simulink model "Proyecto"  (R2023a)
settings: Solver=ode15s  StartTime=0.0  StopTime=10  MaxStep=1E-3  RelTol=1e-3
libraries: fl_lib x16, nesl_utility x6, slpidlib x1
settings Model: LastModifiedBy=DELL
settings DataIOCC: SaveFormat=Array  ReturnWorkspaceOutputs=off  TimeSaveName=t
settings DebuggingCC: AlgebraicLoopMsg=none  ArtificialAlgebraicLoopMsg=none  MaxConsecutiveZCsMsg=none  ModelReferenceExtraNoncontSigs=none  OperatingPointInterfaceChecksumMismatchMsg=none
settings RTWCC: GPUComputeCapability=5.0

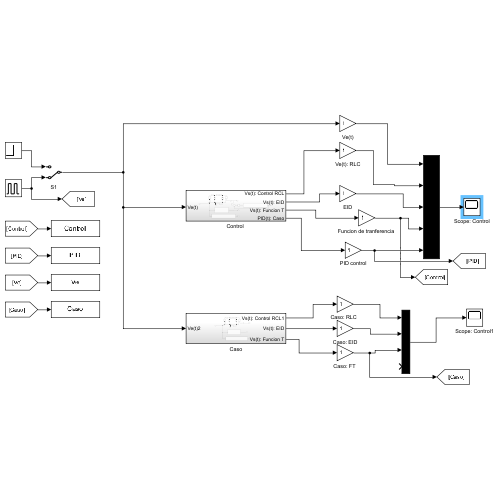
[thumbnail: Simulink's stored preview of the top-level diagram]
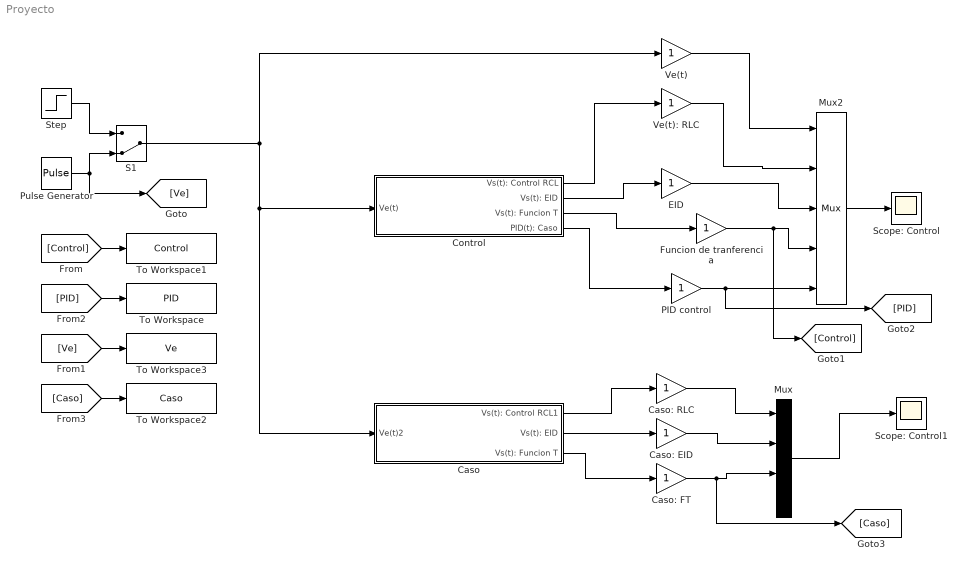
== system Proyecto ==
  Caso : Subsystem
  Caso: EID : Gain
  "Caso: FT " : Gain
  "Caso: RLC  " : Gain
  "Control " : Subsystem
  EID : Gain
  "Funcion de tranferencia " : Gain
  Mux : Mux
  Mux2 : Mux  Inputs=5
  PID control : Gain
  Pulse Generator : DiscretePulseGenerator  PulseType=Time based  Period=10  PulseWidth=10  PhaseDelay=1
  S1 : ManualSwitch  CurrentSetting=0
  Scope: Control : Scope
  Scope: Control1 : Scope
  Step : Step  SampleTime=0
  To Workspace : ToWorkspace  VariableName=PID  SampleTime=-1
  To Workspace1 : ToWorkspace  VariableName=Control  SampleTime=-1
  To Workspace2 : ToWorkspace  VariableName=Caso  SampleTime=-1
  To Workspace3 : ToWorkspace  VariableName=Ve  SampleTime=-1
  Ve(t) : Gain
  Ve(t): RLC : Gain
  wires:
  Mux2/1 -> Scope: Control/1
  Step/1 -> S1/1
  "Control "/1(Vs(t): Control RCL) -> Ve(t): RLC/1
  Pulse Generator/1 -> S1/2, [Ve]
  S1/1 -> Caso/1(Ve(t)2), "Control "/1(Ve(t)), Ve(t)/1
  "Control "/2(Vs(t): EID) -> EID/1
  EID/1 -> Mux2/3
  "Control "/3(Vs(t): Funcion T) -> "Funcion de tranferencia "/1
  "Funcion de tranferencia "/1 -> [Control], Mux2/4
  Ve(t)/1 -> Mux2/1
  Ve(t): RLC/1 -> Mux2/2
  Caso/1(Vs(t): Control RCL1) -> "Caso: RLC  "/1
  Mux/1 -> Scope: Control1/1
  Caso/2(Vs(t): EID) -> Caso: EID/1
  Caso/3(Vs(t): Funcion T) -> "Caso: FT "/1
  "Caso: RLC  "/1 -> Mux/1
  Caso: EID/1 -> Mux/2
  "Caso: FT "/1 -> [Caso], Mux/3
  [Control] -> To Workspace1/1
  [Ve] -> To Workspace3/1
  [PID] -> To Workspace/1
  [Caso] -> To Workspace2/1
  "Control "/4(PID(t): Caso) -> PID control/1
  PID control/1 -> [PID], Mux2/5

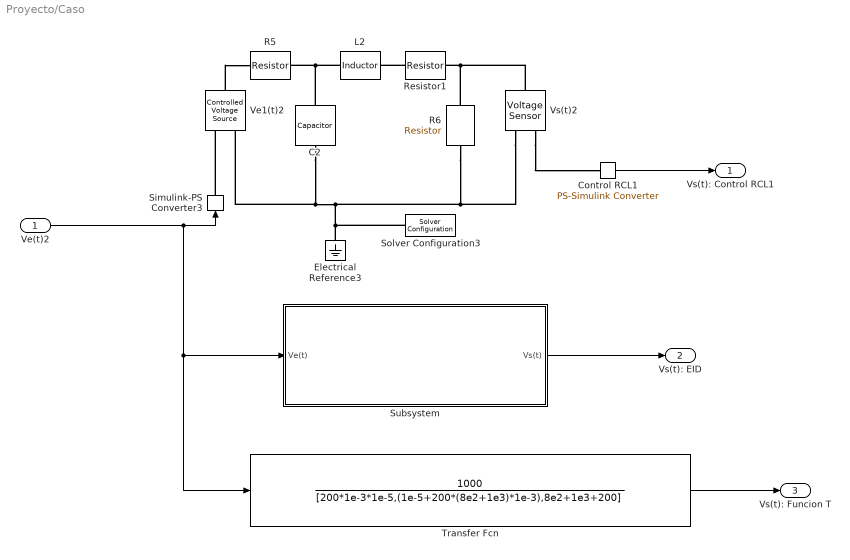
== system Proyecto/Caso ==
  Ve(t)2 : Inport
  C2 : fl_lib/Electrical/Electrical Elements/Capacitor  c=1e-3 F  r=1e-6 Ohm  g=0 1/Ohm  i_specify=off  i_priority=None  i=0 A  i_nominal_specify=off  i_nominal_unit=A  i_nominal_value=1  v_specify=off  v_priority=None  v=0 V  v_nominal_specify=off  v_nominal_unit=V  v_nominal_value=1  vc_specify=off  vc_priority=High  vc=0 V  vc_nominal_specify=off  vc_nominal_unit=V  vc_nominal_value=1
  Control RCL1 : nesl_utility/PS-Simulink Converter  PhysicalDomain=network_engine_domain  SubClassName=ps_output  LeftPortType=input  RightPortType=output  PseudoPeriodic=off  Frequencies=[]  VectorFormat=1-D array  Unit=inherit  AffineConversion=off
  Electrical Reference3 : fl_lib/Electrical/Electrical Elements/Electrical Reference
  L2 : fl_lib/Electrical/Electrical Elements/Inductor  l=1e-5 H  r=0 Ohm  g=1e-9 1/Ohm  i_specify=off  i_priority=None  i=0 A  i_nominal_specify=off  i_nominal_unit=A  i_nominal_value=1  v_specify=off  v_priority=None  v=0 V  v_nominal_specify=off  v_nominal_unit=V  v_nominal_value=1  i_L_specify=off  i_L_priority=High  i_L=0 A  i_L_nominal_specify=off  i_L_nominal_unit=A  i_L_nominal_value=1
  R5 : fl_lib/Electrical/Electrical Elements/Resistor  R=2e2 Ohm  i_specify=off  i_priority=None  i=0 A  i_nominal_specify=off  i_nominal_unit=A  i_nominal_value=1  v_specify=off  v_priority=None  v=0 V  v_nominal_specify=off  v_nominal_unit=V  v_nominal_value=1
  R6 : fl_lib/Electrical/Electrical Elements/Resistor  R=1e3 Ohm  i_specify=off  i_priority=None  i=0 A  i_nominal_specify=off  i_nominal_unit=A  i_nominal_value=1  v_specify=off  v_priority=None  v=0 V  v_nominal_specify=off  v_nominal_unit=V  v_nominal_value=1
  Resistor1 : fl_lib/Electrical/Electrical Elements/Resistor  R=8e2 Ohm  i_specify=off  i_priority=None  i=0 A  i_nominal_specify=off  i_nominal_unit=A  i_nominal_value=1  v_specify=off  v_priority=None  v=0 V  v_nominal_specify=off  v_nominal_unit=V  v_nominal_value=1
  Simulink-PS Converter3 : nesl_utility/Simulink-PS Converter  PhysicalDomain=network_engine_domain  SubClassName=ps_input  LeftPortType=input  RightPortType=output  PseudoPeriodic=off  Frequencies=[]  NoiseDistribution=none  NoiseParameters=[]  Unit=1  AffineConversion=off  FilteringAndDerivatives=provide  SimscapeFilterOrder=1  InputFilterTimeConstant=0.001  UdotUserProvided=0
  Solver Configuration3 : nesl_utility/Solver Configuration  PhysicalDomain=network_engine_domain  SubClassName=solver  LeftPortType=input  RightPortType=generic  Tones=[]  Harmonics=[]  SimulateNoise=off  Profile=off  UseLocalSampling=off  EnableSwitchedLinearOptims=on  FrequencyDomain=off  UseCCode=off  RelTol=0.001  AbsTol=0.001  MinStep=1e-09  ToWorkspace=off  RevertToSquareIcSolve=off  NumHomotopyIterations=100  PhasorMode=off  PhasorModeNumHarmonics=1  ConsistencySolver=NEWTON_XTOL_AFTER_FTOL  IndexReductionMethod=DerivativeReplacement  DoDC=off  ResidualTolerance=1e-09  ConsistencyTolSource=GLOBAL  ConsistencyAbsTol=0.001  ConsistencyRelTol=0.001  ConsistencyTolFactor=0.001  UseLocalSolver=off  LocalSolverChoice=NE_BACKWARD_EULER_ADVANCER  ResolveIndetEquations=on  FunctionEvalNumThread=1  LocalSolverSampleTime=0.001  DoFixedCost=off  MaxNonlinIter=3  MaxModeIter=2  ComputeImpulses=off  ImpulseIterations=2  LinearAlgebra=auto  LinearAlgebraNumThread=0  EquationFormulation=NE_TIME_EF  DelaysMemoryBudget=1024  AutomaticFiltering=on  FilteringTimeConstant=0.001  PartitionStorageMethod=AS_NEEDED  PartitionMemoryBudget=1024  PartitionMethod=ROBUST
  Subsystem : Subsystem
  Transfer Fcn : TransferFcn  Numerator=[1000]  Denominator=[200*1e-3*1e-5,(1e-5+200*(8e2+1e3)*1e-3),8e2+1e3+200]
  Ve1(t)2 : fl_lib/Electrical/Electrical Sources/Controlled Voltage Source
  Vs(t)2 : fl_lib/Electrical/Electrical Sensors/Voltage Sensor
  Vs(t): Control RCL1 : Outport
  Vs(t): EID : Outport  Port=2
  Vs(t): Funcion T : Outport  Port=3
  wires:
  Ve(t)2/1 -> Transfer Fcn/1, Subsystem/1(Ve(t)), Simulink-PS Converter3/1
  Control RCL1/1 -> Vs(t): Control RCL1/1
  Subsystem/1(Vs(t)) -> Vs(t): EID/1
  Transfer Fcn/1 -> Vs(t): Funcion T/1
  connections:
  Ve1(t)2/RConn2 -- Vs(t)2/RConn2 -- R6/LConn1 -- Electrical Reference3/LConn1 -- Solver Configuration3/RConn1 -- C2/RConn1
  R5/LConn1 -- L2/LConn1 -- C2/LConn1
  R6/RConn1 -- Resistor1/RConn1 -- Vs(t)2/LConn1
  Vs(t)2/RConn1 -- Control RCL1/LConn1
  Resistor1/LConn1 -- L2/RConn1
  Simulink-PS Converter3/RConn1 -- Ve1(t)2/RConn1
  Ve1(t)2/LConn1 -- R5/RConn1

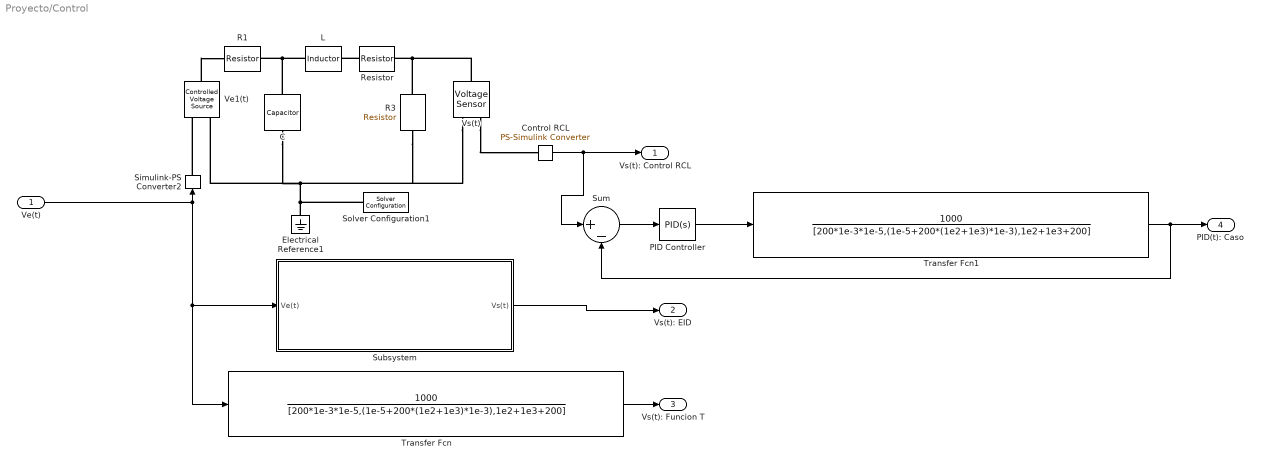
== system Proyecto/Control  ==
  Ve(t) : Inport
  C : fl_lib/Electrical/Electrical Elements/Capacitor  c=1e-3 F  r=1e-6 Ohm  g=0 1/Ohm  i_specify=off  i_priority=None  i=0 A  i_nominal_specify=off  i_nominal_unit=A  i_nominal_value=1  v_specify=off  v_priority=None  v=0 V  v_nominal_specify=off  v_nominal_unit=V  v_nominal_value=1  vc_specify=off  vc_priority=High  vc=0 V  vc_nominal_specify=off  vc_nominal_unit=V  vc_nominal_value=1
  Control RCL : nesl_utility/PS-Simulink Converter  PhysicalDomain=network_engine_domain  SubClassName=ps_output  LeftPortType=input  RightPortType=output  PseudoPeriodic=off  Frequencies=[]  VectorFormat=1-D array  Unit=inherit  AffineConversion=off
  Electrical Reference1 : fl_lib/Electrical/Electrical Elements/Electrical Reference
  L : fl_lib/Electrical/Electrical Elements/Inductor  l=1e-5 H  r=0 Ohm  g=1e-9 1/Ohm  i_specify=off  i_priority=None  i=0 A  i_nominal_specify=off  i_nominal_unit=A  i_nominal_value=1  v_specify=off  v_priority=None  v=0 V  v_nominal_specify=off  v_nominal_unit=V  v_nominal_value=1  i_L_specify=off  i_L_priority=High  i_L=0 A  i_L_nominal_specify=off  i_L_nominal_unit=A  i_L_nominal_value=1
  PID Controller : slpidlib/PID Controller  Controller=PID  Form=Parallel  TimeDomain=Continuous-time  UseExternalTs=off  SampleTime=-1  IntegratorMethod=Forward Euler  FilterMethod=Forward Euler  ControllerParametersSource=internal  P=248.438417147323  I=51942.1111026086  UseKiTs=off  D=0.0387665440418385  N=4312.01473044837  UseFilter=on  TunerSelectOption=Transfer Function Based (PID Tuner App)  InitialConditionSource=internal  InitialConditionForIntegrator=0  InitialConditionForFilter=0  DifferentiatorICPrevScaledInput=0  ExternalReset=none  TrackingMode=off  Kt=1  LimitOutput=off  SatLimitsSource=internal  UpperSaturationLimit=inf  LowerSaturationLimit=-inf  LinearizeAsGain=on  AntiWindupMode=none  Kb=1  LimitIntegrator=off  UpperIntegratorSaturationLimit=inf  LowerIntegratorSaturationLimit=-inf  POutMin=[]  POutMax=[]  IOutMin=[]  IOutMax=[]  DOutMin=[]  DOutMax=[]  NOutMin=[]  NOutMax=[]  SumOutMin=[]  SumOutMax=[]  SaturationOutMin=[]  SaturationOutMax=[]  PParamMin=[]  PParamMax=[]  IParamMin=[]  IParamMax=[]  DParamMin=[]  DParamMax=[]  NParamMin=[]  NParamMax=[]  KbParamMin=[]  KbParamMax=[]  KtParamMin=[]  KtParamMax=[]  KbOutMin=[]  KbOutMax=[]  KtOutMin=[]  KtOutMax=[]  IntegratorOutMin=[]  IntegratorOutMax=[]  FilterOutMin=[]  FilterOutMax=[]  SumI1OutMin=[]  SumI1OutMax=[]  SumI2OutMin=[]  SumI2OutMax=[]  SumI3OutMin=[]  SumI3OutMax=[]  SumI4OutMin=[]  SumI4OutMax=[]  SumDOutMin=[]  SumDOutMax=[]  DifferentiatorOutMin=[]  DifferentiatorOutMax=[]  FilterDiffOutCoefMin=[]  FilterDiffOutCoefMax=[]  ReciprocalOutMin=[]  ReciprocalOutMax=[]  SumDenOutMin=[]  SumDenOutMax=[]  SumNumOutMin=[]  SumNumOutMax=[]  DivideOutMin=[]  DivideOutMax=[]  UdiffTsProdOutMin=[]  UdiffTsProdOutMax=[]  NTsProdOutMin=[]  NTsProdOutMax=[]  UintegralTsProdOutMin=[]  UintegralTsProdOutMax=[]  UngainTsProdOutMin=[]  UngainTsProdOutMax=[]  ClampingZeroOutDataTypeStr=Inherit: Inherit via back propagation  ClampingZeroOutMin=[]  ClampingZeroOutMax=[]  FilterDenConstantOutDataTypeStr=Inherit: Inherit via back propagation  FilterDenConstantOutMin=[]  FilterDenConstantOutMax=[]  PCopyOutDataTypeStr=Inherit: Inherit via back propagation  PCopyOutMin=[]  PCopyOutMax=[]  NCopyOutDataTypeStr=Inherit: Inherit via back propagation  NCopyOutMin=[]  NCopyOutMax=[]  IntegratorContinuousStateAttributes=''  IntegratorStateMustResolveToSignalObject=off  IntegratorRTWStateStorageClass=Auto  FilterContinuousStateAttributes=''  FilterStateMustResolveToSignalObject=off  FilterRTWStateStorageClass=Auto  ParallelPVariant=InternalParameters  IdealPVariant=Disabled  IVariant=InternalParameters  DVariant=InternalParameters  IntegratorVariant=Continuous  SatVariant=Disabled  AWVariant=Passthrough  PCopyVariant=Disabled  TRVariant=Disabled  FdbkBlocksVariant=Forward  IdealPFdbkVariant=Disabled  SatFdbkVariant=Disabled  DerivativeFilterVariant=ContFilter  NVariant=InternalParameters  NCopyVariant=Disabled  FilterICVariant=InternalICsFilter  IntegratorICVariant=InternalICs  ExternalResetVariant=Disabled  TRSumVariant=Passthrough  SumFdbkVariant=Disabled  SumVariant=Sum_PID  TsampFilterVariant=InternalTs  TsampNgainVariant=Passthrough  TsampIntegralVariant=Disabled_SignalSpec  ExternalSaturationOutDataTypeStr=Inherit: Same as second input
  R1 : fl_lib/Electrical/Electrical Elements/Resistor  R=2e2 Ohm  i_specify=off  i_priority=None  i=0 A  i_nominal_specify=off  i_nominal_unit=A  i_nominal_value=1  v_specify=off  v_priority=None  v=0 V  v_nominal_specify=off  v_nominal_unit=V  v_nominal_value=1
  R3 : fl_lib/Electrical/Electrical Elements/Resistor  R=1e3 Ohm  i_specify=off  i_priority=None  i=0 A  i_nominal_specify=off  i_nominal_unit=A  i_nominal_value=1  v_specify=off  v_priority=None  v=0 V  v_nominal_specify=off  v_nominal_unit=V  v_nominal_value=1
  Resistor : fl_lib/Electrical/Electrical Elements/Resistor  R=1e2 Ohm  i_specify=off  i_priority=None  i=0 A  i_nominal_specify=off  i_nominal_unit=A  i_nominal_value=1  v_specify=off  v_priority=None  v=0 V  v_nominal_specify=off  v_nominal_unit=V  v_nominal_value=1
  Simulink-PS Converter2 : nesl_utility/Simulink-PS Converter  PhysicalDomain=network_engine_domain  SubClassName=ps_input  LeftPortType=input  RightPortType=output  PseudoPeriodic=off  Frequencies=[]  NoiseDistribution=none  NoiseParameters=[]  Unit=1  AffineConversion=off  FilteringAndDerivatives=provide  SimscapeFilterOrder=1  InputFilterTimeConstant=0.001  UdotUserProvided=0
  Solver Configuration1 : nesl_utility/Solver Configuration  PhysicalDomain=network_engine_domain  SubClassName=solver  LeftPortType=input  RightPortType=generic  Tones=[]  Harmonics=[]  SimulateNoise=off  Profile=off  UseLocalSampling=off  EnableSwitchedLinearOptims=on  FrequencyDomain=off  UseCCode=off  RelTol=0.001  AbsTol=0.001  MinStep=1e-09  ToWorkspace=off  RevertToSquareIcSolve=off  NumHomotopyIterations=100  PhasorMode=off  PhasorModeNumHarmonics=1  ConsistencySolver=NEWTON_XTOL_AFTER_FTOL  IndexReductionMethod=DerivativeReplacement  DoDC=off  ResidualTolerance=1e-09  ConsistencyTolSource=GLOBAL  ConsistencyAbsTol=0.001  ConsistencyRelTol=0.001  ConsistencyTolFactor=0.001  UseLocalSolver=off  LocalSolverChoice=NE_BACKWARD_EULER_ADVANCER  ResolveIndetEquations=on  FunctionEvalNumThread=1  LocalSolverSampleTime=0.001  DoFixedCost=off  MaxNonlinIter=3  MaxModeIter=2  ComputeImpulses=off  ImpulseIterations=2  LinearAlgebra=auto  LinearAlgebraNumThread=0  EquationFormulation=NE_TIME_EF  DelaysMemoryBudget=1024  AutomaticFiltering=on  FilteringTimeConstant=0.001  PartitionStorageMethod=AS_NEEDED  PartitionMemoryBudget=1024  PartitionMethod=ROBUST
  Subsystem : Subsystem
  Sum : Sum  Inputs=|+-
  Transfer Fcn : TransferFcn  Numerator=[1000]  Denominator=[200*1e-3*1e-5,(1e-5+200*(1e2+1e3)*1e-3),1e2+1e3+200]
  Transfer Fcn1 : TransferFcn  Numerator=[1000]  Denominator=[200*1e-3*1e-5,(1e-5+200*(1e2+1e3)*1e-3),1e2+1e3+200]
  Ve1(t) : fl_lib/Electrical/Electrical Sources/Controlled Voltage Source
  Vs(t) : fl_lib/Electrical/Electrical Sensors/Voltage Sensor
  Vs(t): Control RCL : Outport
  Vs(t): EID : Outport  Port=2
  Vs(t): Funcion T : Outport  Port=3
  PID(t): Caso : Outport  Port=4
  wires:
  Ve(t)/1 -> Transfer Fcn/1, Subsystem/1(Ve(t)), Simulink-PS Converter2/1
  Control RCL/1 -> Sum/1, Vs(t): Control RCL/1
  Subsystem/1(Vs(t)) -> Vs(t): EID/1
  Transfer Fcn/1 -> Vs(t): Funcion T/1
  Sum/1 -> PID Controller/1
  PID Controller/1 -> Transfer Fcn1/1
  Transfer Fcn1/1 -> PID(t): Caso/1, Sum/2
  connections:
  Electrical Reference1/LConn1 -- Solver Configuration1/RConn1 -- C/RConn1 -- Ve1(t)/RConn2 -- Vs(t)/RConn2 -- R3/LConn1
  Ve1(t)/LConn1 -- R1/RConn1
  Vs(t)/RConn1 -- Control RCL/LConn1
  Simulink-PS Converter2/RConn1 -- Ve1(t)/RConn1
  C/LConn1 -- L/LConn1 -- R1/LConn1
  R3/RConn1 -- Resistor/RConn1 -- Vs(t)/LConn1
  Resistor/LConn1 -- L/RConn1

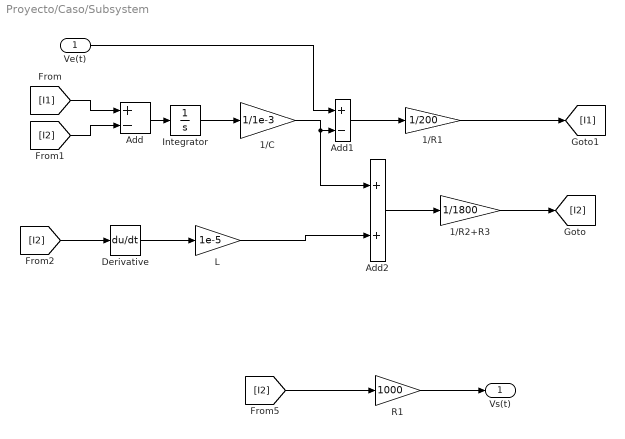
== system Proyecto/Caso/Subsystem ==
  Ve(t) : Inport
  1/C : Gain  Gain=1/1e-3
  1/R1 : Gain  Gain=1/200
  1/R2+R3 : Gain  Gain=1/1800
  Add : Sum  Inputs=+-
  Add1 : Sum  Inputs=+-
  Add2 : Sum
  Derivative : Derivative
  Integrator : Integrator
  L : Gain  Gain=1e-5
  R1 : Gain  Gain=1000
  Vs(t) : Outport
  wires:
  [I1] -> Add/1
  [I2] -> Add/2
  Add/1 -> Integrator/1
  Ve(t)/1 -> Add1/1
  Add1/1 -> 1/R1/1
  [I2] -> Derivative/1
  Add2/1 -> 1/R2+R3/1
  1/R1/1 -> [I1]
  [I2] -> R1/1
  R1/1 -> Vs(t)/1
  1/R2+R3/1 -> [I2]
  1/C/1 -> Add2/1, Add1/2
  Integrator/1 -> 1/C/1
  L/1 -> Add2/2
  Derivative/1 -> L/1

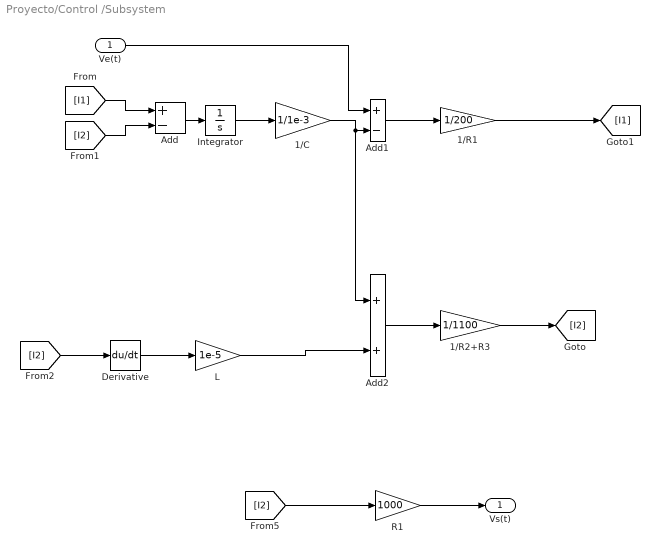
== system Proyecto/Control /Subsystem ==
  Ve(t) : Inport
  1/C : Gain  Gain=1/1e-3
  1/R1 : Gain  Gain=1/200
  1/R2+R3 : Gain  Gain=1/1100
  Add : Sum  Inputs=+-
  Add1 : Sum  Inputs=+-
  Add2 : Sum
  Derivative : Derivative
  Integrator : Integrator
  L : Gain  Gain=1e-5
  R1 : Gain  Gain=1000
  Vs(t) : Outport
  wires:
  [I1] -> Add/1
  [I2] -> Add/2
  Add/1 -> Integrator/1
  Ve(t)/1 -> Add1/1
  Add1/1 -> 1/R1/1
  [I2] -> Derivative/1
  Add2/1 -> 1/R2+R3/1
  1/R1/1 -> [I1]
  [I2] -> R1/1
  R1/1 -> Vs(t)/1
  1/R2+R3/1 -> [I2]
  1/C/1 -> Add2/1, Add1/2
  Integrator/1 -> 1/C/1
  L/1 -> Add2/2
  Derivative/1 -> L/1
